simulink model "closed_loop_load_curr"  (R2024b)
settings: Solver=FixedStepAuto  StartTime=0.0  StopTime=4  RelTol=1e-3
libraries: spsCurrentMeasurementLib x7, spsVoltageMeasurementLib x6, spsSeriesRLCBranchLib x3, spsControlledCurrentSourceLib x1, spsDCVoltageSourceLib x1, spsDiodeLib x1, spsMosfetLib x1, slpidlib x1, simulink x1, SignalEditorBlockLib x1, sps_lib x1
settings Model: Creator=manas  LastModifiedBy=manas

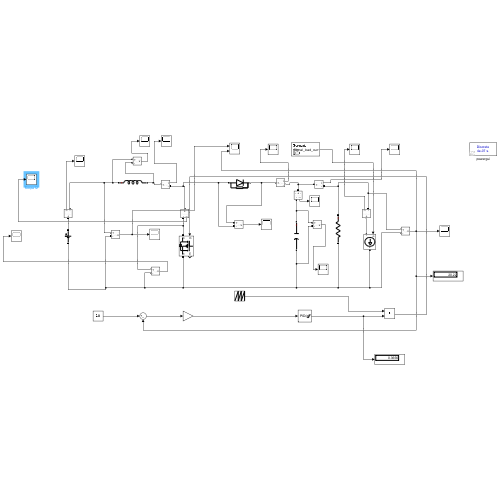
[thumbnail: Simulink's stored preview of the top-level diagram]
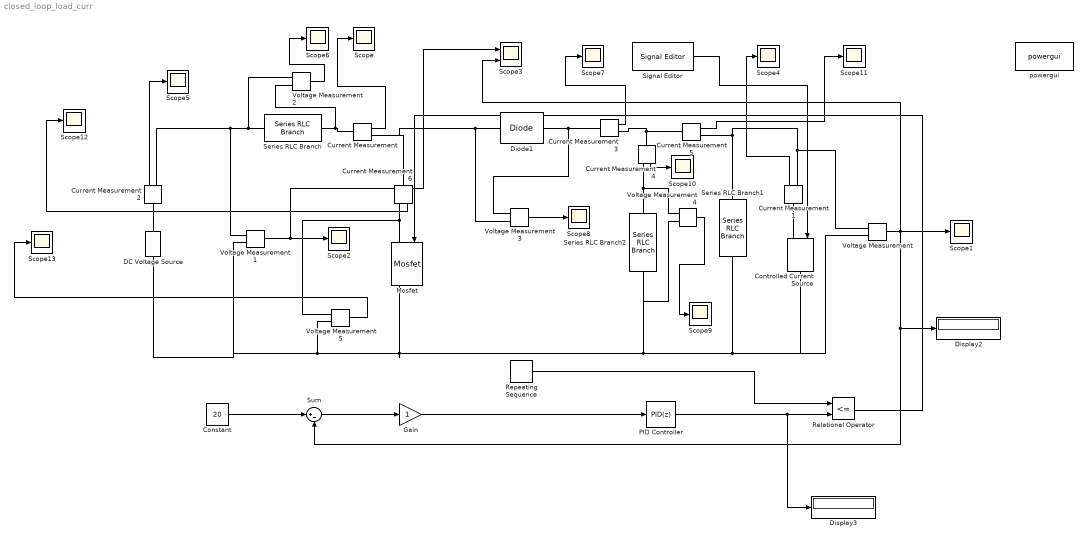
== system closed_loop_load_curr ==
  Constant : Constant  Value=20
  Controlled Current Source : spsControlledCurrentSourceLib/Controlled Current Source  Initialize=on  Source_Type=AC  Amplitude=0  Phase=0  Frequency=0  Measurements=None
  Current Measurement{,1..6} (7 alike) : spsCurrentMeasurementLib/Current Measurement  PhasorSimulation=off  OutputType=Complex  PSBequivalent=0
  DC Voltage Source : spsDCVoltageSourceLib/DC Voltage Source  Amplitude=12  Measurements=None
  Diode1 : spsDiodeLib/Diode  Ron=0.001  Lon=0  Vf=0.8  IC=0  UseSnubber=0  Rs=500  Cs=250e-9  Measurements=off
  Display2 : Display
  Display3 : Display
  Gain : Gain
  Mosfet : spsMosfetLib/Mosfet  Ron=0.1  Lon=0  Rd=0.01  Vfd=0  IC=0  Rs=1e5  Cs=inf  Measurements=on
  PID Controller : slpidlib/PID Controller  Controller=PID  Form=Parallel  TimeDomain=Discrete-time  UseExternalTs=off  SampleTime=-1  IntegratorMethod=Forward Euler  FilterMethod=Forward Euler  ControllerParametersSource=internal  P=0.00534  I=4  UseKiTs=off  D=1e-5  UseExternalDerivativeSource=off  N=20000  UseFilter=on  TunerSelectOption=Transfer Function Based (PID Tuner App)  InitialConditionSource=internal  InitialConditionForIntegrator=0.5  InitialConditionForFilter=0.1  DifferentiatorICPrevScaledInput=0  ExternalReset=none  TrackingMode=off  Kt=1  LimitOutput=on  SatLimitsSource=internal  UpperSaturationLimit=0.9  LowerSaturationLimit=0.1  LinearizeAsGain=on  AntiWindupMode=none  Kb=1  LimitIntegrator=on  UpperIntegratorSaturationLimit=inf  LowerIntegratorSaturationLimit=-inf  POutMin=[]  POutMax=[]  IOutMin=[]  IOutMax=[]  DOutMin=[]  DOutMax=[]  NOutMin=[]  NOutMax=[]  SumOutMin=[]  SumOutMax=[]  SaturationOutMin=[]  SaturationOutMax=[]  PParamMin=[]  PParamMax=[]  IParamMin=[]  IParamMax=[]  DParamMin=[]  DParamMax=[]  NParamMin=[]  NParamMax=[]  KbParamMin=[]  KbParamMax=[]  KtParamMin=[]  KtParamMax=[]  KbOutMin=[]  KbOutMax=[]  KtOutMin=[]  KtOutMax=[]  IntegratorOutMin=[]  IntegratorOutMax=[]  FilterOutMin=[]  FilterOutMax=[]  SumI1OutMin=[]  SumI1OutMax=[]  SumI2OutMin=[]  SumI2OutMax=[]  SumI3OutMin=[]  SumI3OutMax=[]  SumI4OutMin=[]  SumI4OutMax=[]  SumDOutMin=[]  SumDOutMax=[]  DifferentiatorOutMin=[]  DifferentiatorOutMax=[]  FilterDiffOutCoefMin=[]  FilterDiffOutCoefMax=[]  ReciprocalOutMin=[]  ReciprocalOutMax=[]  SumDenOutMin=[]  SumDenOutMax=[]  SumNumOutMin=[]  SumNumOutMax=[]  DivideOutMin=[]  DivideOutMax=[]  UdiffTsProdOutMin=[]  UdiffTsProdOutMax=[]  NTsProdOutMin=[]  NTsProdOutMax=[]  UintegralTsProdOutMin=[]  UintegralTsProdOutMax=[]  UngainTsProdOutMin=[]  UngainTsProdOutMax=[]  ClampingZeroOutDataTypeStr=Inherit: Inherit via back propagation  ClampingZeroOutMin=[]  ClampingZeroOutMax=[]  FilterDenConstantOutDataTypeStr=Inherit: Inherit via back propagation  FilterDenConstantOutMin=[]  FilterDenConstantOutMax=[]  PCopyOutDataTypeStr=Inherit: Inherit via back propagation  PCopyOutMin=[]  PCopyOutMax=[]  NCopyOutDataTypeStr=Inherit: Inherit via back propagation  NCopyOutMin=[]  NCopyOutMax=[]  IntegratorContinuousStateAttributes=''  IntegratorStateMustResolveToSignalObject=off  IntegratorRTWStateStorageClass=Auto  FilterContinuousStateAttributes=''  FilterStateMustResolveToSignalObject=off  FilterRTWStateStorageClass=Auto  ParallelPVariant=InternalParameters  IdealPVariant=Disabled  IVariant=InternalParameters  DVariant=InternalParameters  IntegratorVariant=Discrete  SatVariant=Enabled  AWVariant=Passthrough  PCopyVariant=Disabled  TRVariant=Disabled  FdbkBlocksVariant=Forward  IdealPFdbkVariant=Disabled  SatFdbkVariant=Disabled  DerivativeFilterVariant=ForwardEulerFilter  NVariant=InternalParameters  NCopyVariant=Disabled  FilterICVariant=InternalICsFilter  IntegratorICVariant=InternalICs  ExternalResetVariant=Disabled  TRSumVariant=Passthrough  SumFdbkVariant=Disabled  SumVariant=Sum_PID  TsampFilterVariant=InternalTs  TsampNgainVariant=Passthrough  TsampIntegralVariant=Disabled_SignalSpec  ExternalSaturationOutDataTypeStr=Inherit: Same as second input  DerivativeSourceVariant=ErrorSignal  PreIntVariant=InternalPreInt
  Relational Operator : RelationalOperator  Operator=<=  OutDataTypeStr=boolean  RndMeth=Simplest  InputSameDT=off
  Repeating Sequence : simulink/Sources/Repeating Sequence  rep_seq_t=[0 0.00004]  rep_seq_y=[0 1]
  Scope{,1..2,4..13} (13 alike) : Scope
  Scope3 : Scope  NumInputPorts=2
  Series RLC Branch : spsSeriesRLCBranchLib/Series RLC Branch  LConnTagsString=__new0  RConnTagsString=__new0  BranchType=L  Resistance=1  Inductance=74.6e-6  SetiL0=off  InitialCurrent=0  Capacitance=1e-6  Setx0=off  InitialVoltage=0  Measurements=None
  Series RLC Branch1 : spsSeriesRLCBranchLib/Series RLC Branch  LConnTagsString=__new0  RConnTagsString=__new0  BranchType=R  Resistance=2  Inductance=74.6e-6  SetiL0=off  InitialCurrent=0  Capacitance=1e-6  Setx0=off  InitialVoltage=0  Measurements=None
  Series RLC Branch2 : spsSeriesRLCBranchLib/Series RLC Branch  LConnTagsString=__new0  RConnTagsString=__new0  BranchType=C  Resistance=1  Inductance=1e-3  SetiL0=off  InitialCurrent=0  Capacitance=400e-6  Setx0=off  InitialVoltage=0  Measurements=None
  Signal Editor : SignalEditorBlockLib/Signal Editor  FileName=C:\Users\manas\OneDrive\Desktop\bc_\signal_editor_load_curr (1).mat  ActiveScenario=Scenario  ActiveSignal=Signal_load_curr  IsBus=off  OutputBusObjectStr=Bus: BusObject  SampleTime=0  Interpolate=off  ZeroCross=off  OutputAfterFinalValue=Setting to zero  Unit=inherit  PreserveSignalName=on  ApplySigPropsToAllScenarios=on  ApplySigPropsToAllSignals=off
  Sum : Sum  Inputs=|+-
  Voltage Measurement{,1..5} (6 alike) : spsVoltageMeasurementLib/Voltage Measurement  PhasorSimulation=off  OutputType=Complex  PSBequivalent=0
  powergui : sps_lib/powergui  Priority=1  SimulationMode=Discrete  SampleTime=0.4e-6  frequency=60  Iterations=50  frequencyindice=0  Pbase=100e6  ErrMax=1e-4  UnitsV=kV  UnitsW=MW  buscounter=0  FunctionMessages=off  echomessages=off  EnableUseOfTLC=off  CurrentSourceSwitches=off  DisableSnubberDevices=off  DisableRonSwitches=off  DisableVfSwitches=off  DisplayEquations=off  AutomaticDiscreteSolvers=off  SolverType=Tustin/Backward Euler (TBE)  Interpol=off  ExternalGateDelay=off  methode=off  Ts=100  x0status=blocks  SPID=on  SwTol=0  HookPort=off  NonlinearTolerance=1e-4  nMaxIteration=100  ContinueOnMaxIteration=off  RestoreLinks=warning  ResistiveCurrentMeasurement=off  Frange=[0:2:500]  Ylog=off  Xlog=on  ShowGrid=off  save=off  variable=ZData  structure=0  ZoomFFT=off  StartTime=0.0  cycles=1  DisplayStyle=1  fundamental=60  FreqAxis=off  MaxFrequency=1000  frequencyindicesteady=1  RmsSteady=1  display=off
  wires:
  Sum/1 -> Gain/1
  Current Measurement/1 -> Scope/1
  Voltage Measurement1/1 -> Scope2/1, Scope3/1
  PID Controller/1 -> Display3/1, Relational Operator/2
  Relational Operator/1 -> Mosfet/1
  Constant/1 -> Sum/1
  Gain/1 -> PID Controller/1
  Voltage Measurement/1 -> Display2/1, Sum/2, Scope1/1, Scope3/2
  Repeating Sequence/1 -> Relational Operator/1
  Current Measurement1/1 -> Scope4/1
  Signal Editor/1 -> Controlled Current Source/1
  Current Measurement2/1 -> Scope5/1
  Voltage Measurement2/1 -> Scope6/1
  Current Measurement3/1 -> Scope7/1
  Voltage Measurement3/1 -> Scope8/1
  Voltage Measurement4/1 -> Scope9/1
  Current Measurement4/1 -> Scope10/1
  Current Measurement5/1 -> Scope11/1
  Voltage Measurement5/1 -> Scope13/1
  Current Measurement6/1 -> Scope12/1
  connections:
  Mosfet/RConn1 -- Voltage Measurement5/LConn2 -- DC Voltage Source/LConn1 -- Voltage Measurement1/LConn2 -- Series RLC Branch2/RConn1 -- Voltage Measurement4/LConn2 -- Voltage Measurement/LConn2 -- Controlled Current Source/RConn1 -- Series RLC Branch1/RConn1
  Series RLC Branch1/LConn1 -- Current Measurement1/RConn1 -- Voltage Measurement/LConn1 -- Current Measurement5/RConn1
  Mosfet/LConn1 -- Current Measurement6/RConn1 -- Voltage Measurement5/LConn1
  Voltage Measurement1/LConn1 -- Voltage Measurement2/LConn1 -- Series RLC Branch/LConn1 -- Current Measurement2/RConn1
  Series RLC Branch/RConn1 -- Voltage Measurement2/LConn2 -- Current Measurement/LConn1
  Current Measurement1/LConn1 -- Controlled Current Source/LConn1
  Current Measurement2/LConn1 -- DC Voltage Source/RConn1
  Current Measurement3/LConn1 -- Voltage Measurement3/LConn1 -- Diode1/RConn1
  Series RLC Branch2/LConn1 -- Current Measurement4/RConn1 -- Voltage Measurement4/LConn1
  Current Measurement3/RConn1 -- Current Measurement5/LConn1 -- Current Measurement4/LConn1
  Voltage Measurement3/LConn2 -- Current Measurement6/LConn1 -- Current Measurement/RConn1 -- Diode1/LConn1
